simulink model "quadcopter_ex04_wind_test"  (R2025b)
settings: Solver=ode23t  StartTime=0.0  StopTime=timespot_spl(end)+2  FixedStep=0.01  MaxStep=1e-2  RelTol=1e-3  AbsTol=1e-3
PreLoadFcn:
  | [waypoints, timespot_spl, spline_data, spline_yaw, wayp_path_vis] = quadcopter_package_select_trajectory(2,true);
  | disp('Loaded path 2, round trip');
model workspace (MATLAB code in the model file):
  | load('xy_data_membrane.mat');
values from neighbouring files (symbols this model uses):
  wind_speed = 12    [quadcopter_ex04_wind_test_code.m]
undefined symbols (not defined in the file or in its folder): air_rho, battery_capacity, drone_leg, filtD_altitude, filtD_attitude, filtD_motor, filtD_position, filtD_yaw, filtM_altitude, filtM_attitude, filtM_position, filtM_yaw, filtSpd_motor, kd_altitude, kd_attitude, kd_motor, kd_position, kd_yaw, ki_altitude, ki_attitude, ki_motor, ki_position, ki_yaw, kp_altitude, kp_attitude, kp_motor, kp_position, kp_yaw, limit_altitude, limit_attitude, limit_motor, limit_yaw, pkgDensity, pkgSize, planedepth, pos2attitude, propeller, qc_motor, qd_area, qd_drag, spline_data, spline_yaw, timespot_spl, waypoints, X, Y, Z
libraries: sm_lib x77, nesl_utility x30, fl_lib x13, slpidlib x9, quadcopter_library x6, ee_lib x4, simulink x2, batteryecm_lib x1
(part 2 of 4)

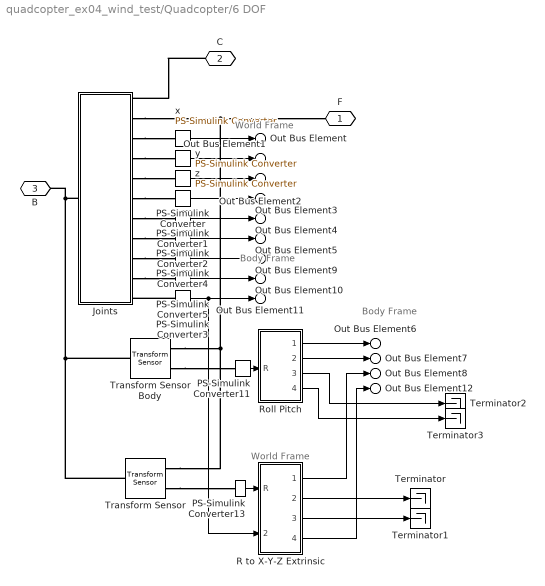
== system quadcopter_ex04_wind_test/Quadcopter/6 DOF ==
  note: Body Frame
  note: World Frame
  note: World Frame
  note: Body Frame
  Joints : Subsystem
  PS-Simulink Converter{,1..2,4..5} (5 alike) : nesl_utility/PS-Simulink Converter  PhysicalDomain=network_engine_domain  SubClassName=ps_output  LeftPortType=input  RightPortType=output  PseudoPeriodic=off  Frequencies=[]  VectorFormat=1-D array  Unit=inherit  AffineConversion=off
  PS-Simulink Converter11 : nesl_utility/PS-Simulink Converter  PhysicalDomain=network_engine_domain  SubClassName=ps_output  LeftPortType=input  RightPortType=output  PseudoPeriodic=off  Frequencies=[]  VectorFormat=1-D array  Unit=1  AffineConversion=off
  PS-Simulink Converter13 : nesl_utility/PS-Simulink Converter  PhysicalDomain=network_engine_domain  SubClassName=ps_output  LeftPortType=input  RightPortType=output  PseudoPeriodic=off  Frequencies=[]  VectorFormat=1-D array  Unit=1  AffineConversion=off
  PS-Simulink Converter3 : nesl_utility/PS-Simulink Converter  PhysicalDomain=network_engine_domain  SubClassName=ps_output  LeftPortType=input  RightPortType=output  PseudoPeriodic=off  Frequencies=[]  VectorFormat=1-D array  Unit=1  AffineConversion=off
  R to X-Y-Z Extrinsic : Subsystem  mask(Rotation Matrix to X-Y-Z Extrinsic){}
      mask help: Computes roll / pitch / yaw values assuming they correspond to X, Y, and Z rotations, applied in that order and using extrinsic rotations (rotations applied about the fixed axes of the base frame). Does not handle case where Y (pitch) rotation is +/-90 degrees.
  Roll Pitch : Subsystem
  Terminator{,1..3} (4 alike) : Terminator
  Transform Sensor : sm_lib/Frames and Transforms/Transform Sensor  MeasurementFrame=World  RotationSequence=XYX  SenseAngle=off  SenseAxis=off  SenseQ=off  SenseR=on  SenseRotationSequence=off  SenseOmegaX=off  SenseOmegaY=off  SenseOmegaZ=off  SenseOmega=off  SenseQDot=off  SenseRDot=off  SenseRotationSequenceDot=off  SenseAlphaX=off  SenseAlphaY=off  SenseAlphaZ=off  SenseAlpha=off  SenseQDDot=off  SenseRDDot=off  SenseX=off  SenseY=off  SenseZ=off  SenseXYZ=off  SenseRad=off  SenseAzim=off  SenseDist=off  SenseInc=off  SenseXDot=off  SenseYDot=off  SenseZDot=off  SenseXYZDot=off  SenseRadDot=off  SenseAzimDot=off  SenseDistDot=off  SenseIncDot=off  SenseXDDot=off  SenseYDDot=off  SenseZDDot=off  SenseXYZDDot=off  SenseRadDDot=off  SenseAzimDDot=off  SenseDistDDot=off  SenseIncDDot=off
  Transform Sensor Body : sm_lib/Frames and Transforms/Transform Sensor  MeasurementFrame=NonRotatingFollower  RotationSequence=XYX  SenseAngle=off  SenseAxis=off  SenseQ=off  SenseR=on  SenseRotationSequence=off  SenseOmegaX=off  SenseOmegaY=off  SenseOmegaZ=off  SenseOmega=off  SenseQDot=off  SenseRDot=off  SenseRotationSequenceDot=off  SenseAlphaX=off  SenseAlphaY=off  SenseAlphaZ=off  SenseAlpha=off  SenseQDDot=off  SenseRDDot=off  SenseX=off  SenseY=off  SenseZ=off  SenseXYZ=off  SenseRad=off  SenseAzim=off  SenseDist=off  SenseInc=off  SenseXDot=off  SenseYDot=off  SenseZDot=off  SenseXYZDot=off  SenseRadDot=off  SenseAzimDot=off  SenseDistDot=off  SenseIncDot=off  SenseXDDot=off  SenseYDDot=off  SenseZDDot=off  SenseXYZDDot=off  SenseRadDDot=off  SenseAzimDDot=off  SenseDistDDot=off  SenseIncDDot=off
  x : nesl_utility/PS-Simulink Converter  PhysicalDomain=network_engine_domain  SubClassName=ps_output  LeftPortType=input  RightPortType=output  PseudoPeriodic=off  Frequencies=[]  VectorFormat=1-D array  Unit=1  AffineConversion=off
  y : nesl_utility/PS-Simulink Converter  PhysicalDomain=network_engine_domain  SubClassName=ps_output  LeftPortType=input  RightPortType=output  PseudoPeriodic=off  Frequencies=[]  VectorFormat=1-D array  Unit=1  AffineConversion=off
  z : nesl_utility/PS-Simulink Converter  PhysicalDomain=network_engine_domain  SubClassName=ps_output  LeftPortType=input  RightPortType=output  PseudoPeriodic=off  Frequencies=[]  VectorFormat=1-D array  Unit=1  AffineConversion=off
  F : PMIOPort  Side=Left
  C : PMIOPort  Port=2  Side=Left
  B : PMIOPort  Port=3  Side=Left
  Out Bus Element : Outport  PortName=m  Element=px
  Out Bus Element1 : Outport  PortName=m  Element=vx
  Out Bus Element2 : Outport  PortName=m  Element=py
  Out Bus Element3 : Outport  PortName=m  Element=vy
  Out Bus Element4 : Outport  PortName=m  Element=pz
  Out Bus Element5 : Outport  PortName=m  Element=vz
  Out Bus Element6 : Outport  PortName=m  Element=roll
  Out Bus Element7 : Outport  PortName=m  Element=pitch
  Out Bus Element8 : Outport  PortName=m  Element=yaw
  Out Bus Element9 : Outport  PortName=m  Element=nRoll
  Out Bus Element10 : Outport  PortName=m  Element=nPitch
  Out Bus Element11 : Outport  PortName=m  Element=nYaw
  Out Bus Element12 : Outport  PortName=m  Element=yawWr
  wires:
  x/1 -> Out Bus Element/1
  y/1 -> Out Bus Element1/1
  R to X-Y-Z Extrinsic/1(yaw) -> Out Bus Element8/1
  PS-Simulink Converter1/1 -> Out Bus Element4/1
  PS-Simulink Converter2/1 -> Out Bus Element5/1
  z/1 -> Out Bus Element2/1
  PS-Simulink Converter/1 -> Out Bus Element3/1
  PS-Simulink Converter11/1 -> Roll Pitch/1(R)
  Roll Pitch/1(aRoll) -> Out Bus Element6/1
  Roll Pitch/2(aPitch) -> Out Bus Element7/1
  R to X-Y-Z Extrinsic/3(roll) -> Terminator1/1
  R to X-Y-Z Extrinsic/2(pitch) -> Terminator/1
  PS-Simulink Converter13/1 -> R to X-Y-Z Extrinsic/1(R)
  Roll Pitch/3(nRoll) -> Terminator2/1
  Roll Pitch/4(nPitch) -> Terminator3/1
  PS-Simulink Converter3/1 -> R to X-Y-Z Extrinsic/2(nYaw), Out Bus Element11/1
  PS-Simulink Converter4/1 -> Out Bus Element9/1
  PS-Simulink Converter5/1 -> Out Bus Element10/1
  R to X-Y-Z Extrinsic/4(yawWr) -> Out Bus Element12/1
  connections:
  Joints/RConn2 -- Transform Sensor/RConn1 -- Transform Sensor Body/RConn1 -- F/RConn1
  Joints/RConn3 -- x/LConn1
  Joints/RConn4 -- y/LConn1
  Transform Sensor Body/LConn1 -- Transform Sensor/LConn1 -- B/RConn1 -- Joints/LConn1
  Joints/RConn5 -- z/LConn1
  Joints/RConn6 -- PS-Simulink Converter/LConn1
  Joints/RConn7 -- PS-Simulink Converter1/LConn1
  Joints/RConn8 -- PS-Simulink Converter2/LConn1
  C/RConn1 -- Joints/RConn1
  Transform Sensor Body/RConn2 -- PS-Simulink Converter11/LConn1
  Transform Sensor/RConn2 -- PS-Simulink Converter13/LConn1
  PS-Simulink Converter3/LConn1 -- Joints/RConn11
  Joints/RConn9 -- PS-Simulink Converter4/LConn1
  Joints/RConn10 -- PS-Simulink Converter5/LConn1

== system quadcopter_ex04_wind_test/Quadcopter/Body ==
  " Arm2" : sm_lib/Body Elements/File Solid  ExtGeomFileName=quadcopter_drone_arm.stp  UnitType=FromFile  ExtGeomFileUnits=m  StepReaderType=HEX  ExportConvexHullGeometry=off  InertiaType=Custom  BasedOnType=Density  Density=1  DensityUnits=g/cm^3  Mass=0.0589152  MassUnits=kg  CenterOfMass=[-4.85019e-05, -0.00435236, -0.00536926]  CenterOfMassUnits=m  MomentsOfInertia=[0.000263222, 0.000260855, 1.23093e-05]  MomentsOfInertiaUnits=kg*m^2  ProductsOfInertia=[1.89459e-06, 5.49897e-08, 2.10429e-08]  ProductsOfInertiaUnits=kg*m^2  GraphicType=FromGeometry  MarkerShape=Sphere  MarkerSize=10  GraphicVisPropType=SimpleVisualProperties  GraphicDiffuseColor=[1.0 0.0 0.2]  GraphicOpacity=1.0  GraphicSpecularColor=[0.5 0.5 0.5 1.0]  GraphicAmbientColor=[0.15 0.15 0.15 1.0]  GraphicEmissiveColor=[0.0 0.0 0.0 1.0]  GraphicShininess=75  DoExposeReferenceFrame=off  SerializedFrames=<Frames><Frame><Id>Frame1</Id><Value><Name>port</Name><Origin><Source>GeometricFeature</Source><FeatureName>planar surface 13</FeatureName></Origin><PrimaryAxis><DefinedDirection>-Z</DefinedDirection><Source>ReferenceFrame</Source><SourceDirection>+Z</SourceDirection><FeatureName></FeatureName></PrimaryAxis><SecondaryAxis><DefinedDirection>-X</DefinedDirection><Source>ReferenceFrame</Source><SourceDirection>+X</SourceDirection><FeatureName></FeatureName></SecondaryAxis></Value></Frame><Frame><Id>Frame2</Id><Value><Name>F2</Name><Origin><Source>GeometricFeature</Source><FeatureName>planar surface 4</FeatureName></Origin><PrimaryAxis><DefinedDirection>+Z</DefinedDirection><Source>ReferenceFrame</Source><SourceDirection>+Z</SourceDirection><FeatureName></FeatureName></PrimaryAxis><SecondaryAxis><DefinedDirection>+X</DefinedDirection><Source>ReferenceFrame</Source><SourceDirection>+X</SourceDirection><FeatureName></FeatureName></SecondaryAxis></Value></Frame><Frame><Id>Frame4</Id><Value><Name>Foot</Name><Origin><Source>GeometricFeature</Source><FeatureName>planar surface 62</FeatureName></Origin><PrimaryAxis><DefinedDirection>+Z</DefinedDirection><Source>ReferenceFrame</Source><SourceDirection>+Z</SourceDirection><FeatureName></FeatureName></PrimaryAxis><SecondaryAxis><DefinedDirection>+X</DefinedDirection><Source>ReferenceFrame</Source><SourceDirection>+X</SourceDirection><FeatureName></FeatureName></SecondaryAxis></Value></Frame></Frames>
  " Arm4" : sm_lib/Body Elements/File Solid  ExtGeomFileName=quadcopter_drone_arm.stp  UnitType=FromFile  ExtGeomFileUnits=m  StepReaderType=HEX  ExportConvexHullGeometry=off  InertiaType=Custom  BasedOnType=Density  Density=1  DensityUnits=g/cm^3  Mass=0.0589152  MassUnits=kg  CenterOfMass=[-4.85019e-05, -0.00435236, -0.00536926]  CenterOfMassUnits=m  MomentsOfInertia=[0.000263222, 0.000260855, 1.23093e-05]  MomentsOfInertiaUnits=kg*m^2  ProductsOfInertia=[1.89459e-06, 5.49897e-08, 2.10429e-08]  ProductsOfInertiaUnits=kg*m^2  GraphicType=FromGeometry  MarkerShape=Sphere  MarkerSize=10  GraphicVisPropType=SimpleVisualProperties  GraphicDiffuseColor=[1.0 0.0 0.2]  GraphicOpacity=1.0  GraphicSpecularColor=[0.5 0.5 0.5 1.0]  GraphicAmbientColor=[0.15 0.15 0.15 1.0]  GraphicEmissiveColor=[0.0 0.0 0.0 1.0]  GraphicShininess=75  DoExposeReferenceFrame=off  SerializedFrames=<Frames><Frame><Id>Frame1</Id><Value><Name>port</Name><Origin><Source>GeometricFeature</Source><FeatureName>planar surface 13</FeatureName></Origin><PrimaryAxis><DefinedDirection>-Z</DefinedDirection><Source>ReferenceFrame</Source><SourceDirection>+Z</SourceDirection><FeatureName></FeatureName></PrimaryAxis><SecondaryAxis><DefinedDirection>-X</DefinedDirection><Source>ReferenceFrame</Source><SourceDirection>+X</SourceDirection><FeatureName></FeatureName></SecondaryAxis></Value></Frame><Frame><Id>Frame2</Id><Value><Name>F2</Name><Origin><Source>GeometricFeature</Source><FeatureName>planar surface 4</FeatureName></Origin><PrimaryAxis><DefinedDirection>+Z</DefinedDirection><Source>ReferenceFrame</Source><SourceDirection>+Z</SourceDirection><FeatureName></FeatureName></PrimaryAxis><SecondaryAxis><DefinedDirection>+X</DefinedDirection><Source>ReferenceFrame</Source><SourceDirection>+X</SourceDirection><FeatureName></FeatureName></SecondaryAxis></Value></Frame><Frame><Id>Frame3</Id><Value><Name>Foot</Name><Origin><Source>GeometricFeature</Source><FeatureName>planar surface 62</FeatureName></Origin><PrimaryAxis><DefinedDirection>+Z</DefinedDirection><Source>ReferenceFrame</Source><SourceDirection>+Z</SourceDirection><FeatureName></FeatureName></PrimaryAxis><SecondaryAxis><DefinedDirection>+X</DefinedDirection><Source>ReferenceFrame</Source><SourceDirection>+X</SourceDirection><FeatureName></FeatureName></SecondaryAxis></Value></Frame></Frames>
  Arm1 : sm_lib/Body Elements/File Solid  ExtGeomFileName=quadcopter_drone_arm.stp  UnitType=FromFile  ExtGeomFileUnits=m  StepReaderType=HEX  ExportConvexHullGeometry=off  InertiaType=Custom  BasedOnType=Density  Density=1  DensityUnits=g/cm^3  Mass=0.0589152  MassUnits=kg  CenterOfMass=[-4.85019e-05, -0.00435236, -0.00536926]  CenterOfMassUnits=m  MomentsOfInertia=[0.000263222, 0.000260855, 1.23093e-05]  MomentsOfInertiaUnits=kg*m^2  ProductsOfInertia=[1.89459e-06, 5.49897e-08, 2.10429e-08]  ProductsOfInertiaUnits=kg*m^2  GraphicType=FromGeometry  MarkerShape=Sphere  MarkerSize=10  GraphicVisPropType=SimpleVisualProperties  GraphicDiffuseColor=[1.0 1.0 1.0]  GraphicOpacity=1.0  GraphicSpecularColor=[0.5 0.5 0.5 1.0]  GraphicAmbientColor=[0.15 0.15 0.15 1.0]  GraphicEmissiveColor=[0.0 0.0 0.0 1.0]  GraphicShininess=75  DoExposeReferenceFrame=off  SerializedFrames=<Frames><Frame><Id>Frame1</Id><Value><Name>port</Name><Origin><Source>GeometricFeature</Source><FeatureName>planar surface 13</FeatureName></Origin><PrimaryAxis><DefinedDirection>-Z</DefinedDirection><Source>ReferenceFrame</Source><SourceDirection>+Z</SourceDirection><FeatureName></FeatureName></PrimaryAxis><SecondaryAxis><DefinedDirection>-X</DefinedDirection><Source>ReferenceFrame</Source><SourceDirection>+X</SourceDirection><FeatureName></FeatureName></SecondaryAxis></Value></Frame><Frame><Id>Frame2</Id><Value><Name>F2</Name><Origin><Source>GeometricFeature</Source><FeatureName>planar surface 4</FeatureName></Origin><PrimaryAxis><DefinedDirection>+Z</DefinedDirection><Source>ReferenceFrame</Source><SourceDirection>+Z</SourceDirection><FeatureName></FeatureName></PrimaryAxis><SecondaryAxis><DefinedDirection>+X</DefinedDirection><Source>ReferenceFrame</Source><SourceDirection>+X</SourceDirection><FeatureName></FeatureName></SecondaryAxis></Value></Frame><Frame><Id>Frame3</Id><Value><Name>Foot</Name><Origin><Source>GeometricFeature</Source><FeatureName>planar surface 62</FeatureName></Origin><PrimaryAxis><DefinedDirection>+Z</DefinedDirection><Source>ReferenceFrame</Source><SourceDirection>+Z</SourceDirection><FeatureName></FeatureName></PrimaryAxis><SecondaryAxis><DefinedDirection>+X</DefinedDirection><Source>ReferenceFrame</Source><SourceDirection>+X</SourceDirection><FeatureName></FeatureName></SecondaryAxis></Value></Frame></Frames>
  Arm3 : sm_lib/Body Elements/File Solid  ExtGeomFileName=quadcopter_drone_arm.stp  UnitType=FromFile  ExtGeomFileUnits=m  StepReaderType=HEX  ExportConvexHullGeometry=off  InertiaType=Custom  BasedOnType=Density  Density=1  DensityUnits=g/cm^3  Mass=0.0589152  MassUnits=kg  CenterOfMass=[-4.85019e-05, -0.00435236, -0.00536926]  CenterOfMassUnits=m  MomentsOfInertia=[0.000263222, 0.000260855, 1.23093e-05]  MomentsOfInertiaUnits=kg*m^2  ProductsOfInertia=[1.89459e-06, 5.49897e-08, 2.10429e-08]  ProductsOfInertiaUnits=kg*m^2  GraphicType=FromGeometry  MarkerShape=Sphere  MarkerSize=10  GraphicVisPropType=SimpleVisualProperties  GraphicDiffuseColor=[1.0 1.0 1.0]  GraphicOpacity=1.0  GraphicSpecularColor=[0.5 0.5 0.5 1.0]  GraphicAmbientColor=[0.15 0.15 0.15 1.0]  GraphicEmissiveColor=[0.0 0.0 0.0 1.0]  GraphicShininess=75  DoExposeReferenceFrame=off  SerializedFrames=<Frames><Frame><Id>Frame1</Id><Value><Name>port</Name><Origin><Source>GeometricFeature</Source><FeatureName>planar surface 13</FeatureName></Origin><PrimaryAxis><DefinedDirection>-Z</DefinedDirection><Source>ReferenceFrame</Source><SourceDirection>+Z</SourceDirection><FeatureName></FeatureName></PrimaryAxis><SecondaryAxis><DefinedDirection>-X</DefinedDirection><Source>ReferenceFrame</Source><SourceDirection>+X</SourceDirection><FeatureName></FeatureName></SecondaryAxis></Value></Frame><Frame><Id>Frame2</Id><Value><Name>F2</Name><Origin><Source>GeometricFeature</Source><FeatureName>planar surface 4</FeatureName></Origin><PrimaryAxis><DefinedDirection>+Z</DefinedDirection><Source>ReferenceFrame</Source><SourceDirection>+Z</SourceDirection><FeatureName></FeatureName></PrimaryAxis><SecondaryAxis><DefinedDirection>+X</DefinedDirection><Source>ReferenceFrame</Source><SourceDirection>+X</SourceDirection><FeatureName></FeatureName></SecondaryAxis></Value></Frame><Frame><Id>Frame3</Id><Value><Name>Foot</Name><Origin><Source>GeometricFeature</Source><FeatureName>planar surface 62</FeatureName></Origin><PrimaryAxis><DefinedDirection>+Z</DefinedDirection><Source>ReferenceFrame</Source><SourceDirection>+Z</SourceDirection><FeatureName></FeatureName></PrimaryAxis><SecondaryAxis><DefinedDirection>+X</DefinedDirection><Source>ReferenceFrame</Source><SourceDirection>+X</SourceDirection><FeatureName></FeatureName></SecondaryAxis></Value></Frame></Frames>
  Body : Subsystem
  Legs : Subsystem
  Transform Arm Ref : sm_lib/Frames and Transforms/Rigid Transform  RotationMethod=StandardAxis  FollAlignAxisA=+X  BaseAlignAxisA=+Y  FollAlignAxisB=+Y  BaseAlignAxisB=+Z  RotationStandardAxis=+Z  RotationAngle=45  RotationAngleUnits=deg  RotationArbitraryAxis=[0 0 1]  RotationSequenceAxes=FollowerAxes  RotationSequence=XYX  RotationSequenceAngles=[0 0 0]  RotationSequenceAnglesUnits=deg  RotationMatrix=[1 0 0; 0 1 0; 0 0 1]  Quaternion=[1 0 0 0]  TranslationMethod=Cartesian  TranslationCartesianOffset=[0 0 -26]  TranslationCartesianOffsetUnits=mm  TranslationStandardAxis=+Z  TranslationStandardOffset=0  TranslationStandardOffsetUnits=mm  TranslationROffset=0  TranslationROffsetUnits=m  TranslationThetaOffset=0  TranslationThetaOffsetUnits=deg  TranslationZOffset=0  TranslationZOffsetUnits=m
  Transform Arm1 : sm_lib/Frames and Transforms/Rigid Transform  RotationMethod=RotationSequence  FollAlignAxisA=+X  BaseAlignAxisA=+Y  FollAlignAxisB=+Y  BaseAlignAxisB=+Z  RotationStandardAxis=+Z  RotationAngle=0  RotationAngleUnits=deg  RotationArbitraryAxis=[0 0 1]  RotationSequenceAxes=FollowerAxes  RotationSequence=ZXZ  RotationSequenceAngles=[0 90 0]  RotationSequenceAnglesUnits=deg  RotationMatrix=[1 0 0; 0 1 0; 0 0 1]  Quaternion=[1 0 0 0]  TranslationMethod=Cartesian  TranslationCartesianOffset=[12 58 -38]  TranslationCartesianOffsetUnits=mm  TranslationStandardAxis=+Z  TranslationStandardOffset=0  TranslationStandardOffsetUnits=mm  TranslationROffset=0  TranslationROffsetUnits=m  TranslationThetaOffset=0  TranslationThetaOffsetUnits=deg  TranslationZOffset=0  TranslationZOffsetUnits=m
  Transform Arm2 : sm_lib/Frames and Transforms/Rigid Transform  RotationMethod=RotationSequence  FollAlignAxisA=+X  BaseAlignAxisA=+Y  FollAlignAxisB=+Y  BaseAlignAxisB=+Z  RotationStandardAxis=+Z  RotationAngle=-90  RotationAngleUnits=deg  RotationArbitraryAxis=[0 0 1]  RotationSequenceAxes=FollowerAxes  RotationSequence=ZXZ  RotationSequenceAngles=[-90 90 0]  RotationSequenceAnglesUnits=deg  RotationMatrix=[1 0 0; 0 1 0; 0 0 1]  Quaternion=[1 0 0 0]  TranslationMethod=Cartesian  TranslationCartesianOffset=[58 -12 -38]  TranslationCartesianOffsetUnits=mm  TranslationStandardAxis=+Z  TranslationStandardOffset=0  TranslationStandardOffsetUnits=mm  TranslationROffset=0  TranslationROffsetUnits=m  TranslationThetaOffset=0  TranslationThetaOffsetUnits=deg  TranslationZOffset=0  TranslationZOffsetUnits=m
  Transform Arm3 : sm_lib/Frames and Transforms/Rigid Transform  RotationMethod=RotationSequence  FollAlignAxisA=+X  BaseAlignAxisA=+Y  FollAlignAxisB=+Y  BaseAlignAxisB=+Z  RotationStandardAxis=+Z  RotationAngle=90  RotationAngleUnits=deg  RotationArbitraryAxis=[0 0 1]  RotationSequenceAxes=FollowerAxes  RotationSequence=ZXZ  RotationSequenceAngles=[90 90 0]  RotationSequenceAnglesUnits=deg  RotationMatrix=[1 0 0; 0 1 0; 0 0 1]  Quaternion=[1 0 0 0]  TranslationMethod=Cartesian  TranslationCartesianOffset=[-58 12 -38]  TranslationCartesianOffsetUnits=mm  TranslationStandardAxis=+Z  TranslationStandardOffset=0  TranslationStandardOffsetUnits=mm  TranslationROffset=0  TranslationROffsetUnits=m  TranslationThetaOffset=0  TranslationThetaOffsetUnits=deg  TranslationZOffset=0  TranslationZOffsetUnits=m
  Transform Arm4 : sm_lib/Frames and Transforms/Rigid Transform  RotationMethod=RotationSequence  FollAlignAxisA=+X  BaseAlignAxisA=+Y  FollAlignAxisB=+Y  BaseAlignAxisB=+Z  RotationStandardAxis=+Z  RotationAngle=180  RotationAngleUnits=deg  RotationArbitraryAxis=[0 0 1]  RotationSequenceAxes=FollowerAxes  RotationSequence=ZXZ  RotationSequenceAngles=[180 90 0]  RotationSequenceAnglesUnits=deg  RotationMatrix=[1 0 0; 0 1 0; 0 0 1]  Quaternion=[1 0 0 0]  TranslationMethod=Cartesian  TranslationCartesianOffset=[-12 -58 -38]  TranslationCartesianOffsetUnits=mm  TranslationStandardAxis=+Z  TranslationStandardOffset=0  TranslationStandardOffsetUnits=mm  TranslationROffset=0  TranslationROffsetUnits=m  TranslationThetaOffset=0  TranslationThetaOffsetUnits=deg  TranslationZOffset=0  TranslationZOffsetUnits=m
  P2 : PMIOPort  Side=Right
  "P1 " : PMIOPort  Port=2  Side=Left
  P3 : PMIOPort  Port=3  Side=Left
  P4 : PMIOPort  Port=4  Side=Right
  Ref : PMIOPort  Port=5  Side=Left
  G : PMIOPort  Port=6  Side=Right
  connections:
  Transform Arm4/LConn1 -- Transform Arm1/LConn1 -- Transform Arm3/LConn1 -- Transform Arm Ref/LConn1 -- Transform Arm2/LConn1
  Transform Arm4/RConn1 -- " Arm4"/LConn1
  " Arm2"/RConn1 -- P2/RConn1
  " Arm4"/RConn1 -- P4/RConn1
  Arm3/RConn1 -- P3/RConn1
  " Arm2"/LConn1 -- Transform Arm2/RConn1
  Transform Arm1/RConn1 -- Arm1/LConn1
  Arm1/RConn1 -- "P1 "/RConn1
  Arm3/LConn1 -- Transform Arm3/RConn1
  Legs/RConn1 -- G/RConn1
  Body/RConn1 -- Transform Arm Ref/RConn1
  Ref/RConn1 -- Legs/LConn1 -- Body/LConn1

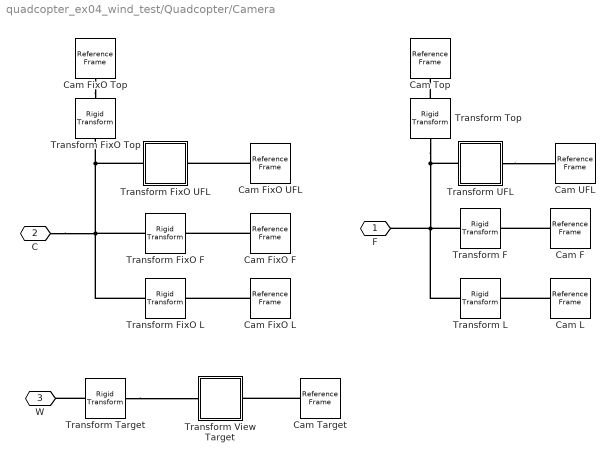
== system quadcopter_ex04_wind_test/Quadcopter/Camera ==
  Cam F : sm_lib/Frames and Transforms/Reference Frame
  Cam FixO F : sm_lib/Frames and Transforms/Reference Frame
  Cam FixO L : sm_lib/Frames and Transforms/Reference Frame
  Cam FixO Top : sm_lib/Frames and Transforms/Reference Frame
  Cam FixO UFL : sm_lib/Frames and Transforms/Reference Frame
  Cam L : sm_lib/Frames and Transforms/Reference Frame
  Cam Target : sm_lib/Frames and Transforms/Reference Frame
  Cam Top : sm_lib/Frames and Transforms/Reference Frame
  Cam UFL : sm_lib/Frames and Transforms/Reference Frame
  Transform Top : sm_lib/Frames and Transforms/Rigid Transform  RotationMethod=RotationSequence  FollAlignAxisA=+X  BaseAlignAxisA=+Y  FollAlignAxisB=+Y  BaseAlignAxisB=+Z  RotationStandardAxis=+Z  RotationAngle=0.0  RotationAngleUnits=deg  RotationArbitraryAxis=[0 0 1]  RotationSequenceAxes=FollowerAxes  RotationSequence=ZYX  RotationSequenceAngles=[0 90 0]  RotationSequenceAnglesUnits=deg  RotationMatrix=[1 0 0; 0 1 0; 0 0 1]  Quaternion=[1 0 0 0]  TranslationMethod=Cartesian  TranslationCartesianOffset=[0 0 1]  TranslationCartesianOffsetUnits=m  TranslationStandardAxis=+Z  TranslationStandardOffset=0  TranslationStandardOffsetUnits=m  TranslationROffset=0  TranslationROffsetUnits=m  TranslationThetaOffset=0  TranslationThetaOffsetUnits=deg  TranslationZOffset=0  TranslationZOffsetUnits=m
  Transform FixO Top : sm_lib/Frames and Transforms/Rigid Transform  RotationMethod=RotationSequence  FollAlignAxisA=+X  BaseAlignAxisA=+Y  FollAlignAxisB=+Y  BaseAlignAxisB=+Z  RotationStandardAxis=+Z  RotationAngle=0.0  RotationAngleUnits=deg  RotationArbitraryAxis=[0 0 1]  RotationSequenceAxes=FollowerAxes  RotationSequence=ZYX  RotationSequenceAngles=[0 90 0]  RotationSequenceAnglesUnits=deg  RotationMatrix=[1 0 0; 0 1 0; 0 0 1]  Quaternion=[1 0 0 0]  TranslationMethod=Cartesian  TranslationCartesianOffset=[0 0 1]  TranslationCartesianOffsetUnits=m  TranslationStandardAxis=+Z  TranslationStandardOffset=0  TranslationStandardOffsetUnits=m  TranslationROffset=0  TranslationROffsetUnits=m  TranslationThetaOffset=0  TranslationThetaOffsetUnits=deg  TranslationZOffset=0  TranslationZOffsetUnits=m
  Transform F : sm_lib/Frames and Transforms/Rigid Transform  RotationMethod=RotationSequence  FollAlignAxisA=+X  BaseAlignAxisA=+Y  FollAlignAxisB=+Y  BaseAlignAxisB=+Z  RotationStandardAxis=+Z  RotationAngle=0.0  RotationAngleUnits=deg  RotationArbitraryAxis=[0 0 1]  RotationSequenceAxes=FollowerAxes  RotationSequence=ZYX  RotationSequenceAngles=[180 0 0]  RotationSequenceAnglesUnits=deg  RotationMatrix=[1 0 0; 0 1 0; 0 0 1]  Quaternion=[1 0 0 0]  TranslationMethod=Cartesian  TranslationCartesianOffset=[1 0 0]  TranslationCartesianOffsetUnits=m  TranslationStandardAxis=+Z  TranslationStandardOffset=0  TranslationStandardOffsetUnits=m  TranslationROffset=0  TranslationROffsetUnits=m  TranslationThetaOffset=0  TranslationThetaOffsetUnits=deg  TranslationZOffset=0  TranslationZOffsetUnits=m
  Transform FixO F : sm_lib/Frames and Transforms/Rigid Transform  RotationMethod=RotationSequence  FollAlignAxisA=+X  BaseAlignAxisA=+Y  FollAlignAxisB=+Y  BaseAlignAxisB=+Z  RotationStandardAxis=+Z  RotationAngle=0.0  RotationAngleUnits=deg  RotationArbitraryAxis=[0 0 1]  RotationSequenceAxes=FollowerAxes  RotationSequence=ZYX  RotationSequenceAngles=[180 0 0]  RotationSequenceAnglesUnits=deg  RotationMatrix=[1 0 0; 0 1 0; 0 0 1]  Quaternion=[1 0 0 0]  TranslationMethod=Cartesian  TranslationCartesianOffset=[1 0 0]  TranslationCartesianOffsetUnits=m  TranslationStandardAxis=+Z  TranslationStandardOffset=0  TranslationStandardOffsetUnits=m  TranslationROffset=0  TranslationROffsetUnits=m  TranslationThetaOffset=0  TranslationThetaOffsetUnits=deg  TranslationZOffset=0  TranslationZOffsetUnits=m
  Transform FixO L : sm_lib/Frames and Transforms/Rigid Transform  RotationMethod=RotationSequence  FollAlignAxisA=+X  BaseAlignAxisA=+Y  FollAlignAxisB=+Y  BaseAlignAxisB=+Z  RotationStandardAxis=+Z  RotationAngle=0.0  RotationAngleUnits=deg  RotationArbitraryAxis=[0 0 1]  RotationSequenceAxes=FollowerAxes  RotationSequence=ZYX  RotationSequenceAngles=[90 0 0]  RotationSequenceAnglesUnits=deg  RotationMatrix=[1 0 0; 0 1 0; 0 0 1]  Quaternion=[1 0 0 0]  TranslationMethod=Cartesian  TranslationCartesianOffset=[0 -1 0]  TranslationCartesianOffsetUnits=m  TranslationStandardAxis=+Z  TranslationStandardOffset=0  TranslationStandardOffsetUnits=m  TranslationROffset=0  TranslationROffsetUnits=m  TranslationThetaOffset=0  TranslationThetaOffsetUnits=deg  TranslationZOffset=0  TranslationZOffsetUnits=m
  Transform FixO UFL : Subsystem  mask{offset_xyz=[0.5 -1 1]}
      mask prompts: offset_xyz "Offset [x y z] (m)"
      mask init:
      | seq_zyx_follower = [atan2d(-offset_xyz(2),-offset_xyz(1)) atan2d(offset_xyz(3),sqrt(offset_xyz(1)^2+offset_xyz(2)^2)) 0];
  Transform L : sm_lib/Frames and Transforms/Rigid Transform  RotationMethod=RotationSequence  FollAlignAxisA=+X  BaseAlignAxisA=+Y  FollAlignAxisB=+Y  BaseAlignAxisB=+Z  RotationStandardAxis=+Z  RotationAngle=0.0  RotationAngleUnits=deg  RotationArbitraryAxis=[0 0 1]  RotationSequenceAxes=FollowerAxes  RotationSequence=ZYX  RotationSequenceAngles=[90 0 0]  RotationSequenceAnglesUnits=deg  RotationMatrix=[1 0 0; 0 1 0; 0 0 1]  Quaternion=[1 0 0 0]  TranslationMethod=Cartesian  TranslationCartesianOffset=[0 -1 0]  TranslationCartesianOffsetUnits=m  TranslationStandardAxis=+Z  TranslationStandardOffset=0  TranslationStandardOffsetUnits=m  TranslationROffset=0  TranslationROffsetUnits=m  TranslationThetaOffset=0  TranslationThetaOffsetUnits=deg  TranslationZOffset=0  TranslationZOffsetUnits=m
  Transform Target : sm_lib/Frames and Transforms/Rigid Transform  RotationMethod=None  FollAlignAxisA=+X  BaseAlignAxisA=+Y  FollAlignAxisB=+Y  BaseAlignAxisB=+Z  RotationStandardAxis=+Z  RotationAngle=0.0  RotationAngleUnits=deg  RotationArbitraryAxis=[0 0 1]  RotationSequenceAxes=FollowerAxes  RotationSequence=ZYX  RotationSequenceAngles=[90 0 0]  RotationSequenceAnglesUnits=deg  RotationMatrix=[1 0 0; 0 1 0; 0 0 1]  Quaternion=[1 0 0 0]  TranslationMethod=Cartesian  TranslationCartesianOffset=[waypoints(1:2,end)' 0 ]  TranslationCartesianOffsetUnits=m  TranslationStandardAxis=+Z  TranslationStandardOffset=0  TranslationStandardOffsetUnits=m  TranslationROffset=0  TranslationROffsetUnits=m  TranslationThetaOffset=0  TranslationThetaOffsetUnits=deg  TranslationZOffset=0  TranslationZOffsetUnits=m
  Transform UFL : Subsystem  mask{offset_xyz=[0.5 -1 1]}
      mask prompts: offset_xyz "Offset [x y z] (m)"
      mask init:
      | seq_zyx_follower = [atan2d(-offset_xyz(2),-offset_xyz(1)) atan2d(offset_xyz(3),sqrt(offset_xyz(1)^2+offset_xyz(2)^2)) 0];
  Transform View Target : Subsystem  mask{offset_xyz=[1.5 -1.5 1]}
      mask prompts: offset_xyz "Offset [x y z] (m)"
      mask init:
      | seq_zyx_follower = [atan2d(-offset_xyz(2),-offset_xyz(1)) atan2d(offset_xyz(3),sqrt(offset_xyz(1)^2+offset_xyz(2)^2)) 0];
  F : PMIOPort  Side=Right
  C : PMIOPort  Port=2  Side=Right
  W : PMIOPort  Port=3  Side=Right
  connections:
  Transform Top/LConn1 -- Transform UFL/LConn1 -- F/RConn1 -- Transform F/LConn1 -- Transform L/LConn1
  C/RConn1 -- Transform FixO L/LConn1 -- Transform FixO F/LConn1 -- Transform FixO UFL/LConn1 -- Transform FixO Top/LConn1
  Cam FixO Top/RConn1 -- Transform FixO Top/RConn1
  Transform Top/RConn1 -- Cam Top/RConn1
  Cam FixO L/RConn1 -- Transform FixO L/RConn1
  Cam L/RConn1 -- Transform L/RConn1
  Cam FixO F/RConn1 -- Transform FixO F/RConn1
  Cam F/RConn1 -- Transform F/RConn1
  Transform UFL/RConn1 -- Cam UFL/RConn1
  Cam FixO UFL/RConn1 -- Transform FixO UFL/RConn1
  Transform Target/LConn1 -- W/RConn1
  Transform Target/RConn1 -- Transform View Target/LConn1
  Cam Target/RConn1 -- Transform View Target/RConn1

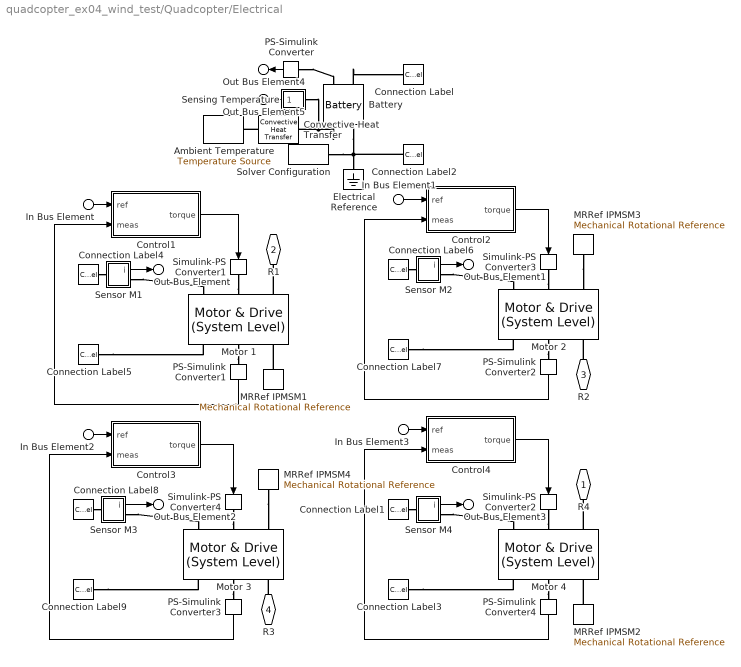
== system quadcopter_ex04_wind_test/Quadcopter/Electrical ==
  In Bus Element : Inport  PortName=cmd  Element=w1
  In Bus Element1 : Inport  PortName=cmd  Element=w2
  In Bus Element2 : Inport  PortName=cmd  Element=w3
  In Bus Element3 : Inport  PortName=cmd  Element=w4
  Ambient Temperature : fl_lib/Thermal/Thermal Sources/Temperature Source  temperature=air_temperature K
  Battery : batteryecm_lib/Battery  Vnom=14 V  prm_dir=1  R1_dis=2 Ohm  R1_ch=2 Ohm  R1=2e-2 Ohm  prm_AH=2  AH=battery_capacity A*hr  V1=11.5 V  AH1=battery_capacity/2 A*hr  prm_R2=1  R2=2000 Ohm  Tmeas=298.15 K  charge_measurement_port=simscape.enum.battery.enable.yes  prm_dyn=1  Rp1=0.005 Ohm  tau1=30 s  Rp2=0.005 Ohm  tau2=30 s  Rp3=0.005 Ohm  tau3=30 s  Rp4=0.005 Ohm  tau4=30 s  Rp5=0.005 Ohm  tau5=30 s  prm_fade=1  N_fade=100  AH_fade=45 A*hr  R1_fade=2.02 Ohm  R1_ch_fade=2.02 Ohm  V1_fade=10.35 V  prm_age=1  prm_age_OCV=1  OCV_age=0.9  SOC_age=60  Tmeas_age=298.15 K  delta_time_age_vec=[0] d  temperature_age_vec=[273] K  OCV_scaling_age=2.2134e6  OCV_offset_age=1.632e6  temp_exp_age=0.515833569 V  t_exp_age=0.75  Vnom_T2=12 V  R1_T2=2e-2 Ohm  R1_T2_dis=2.2 Ohm  R1_T2_ch=2.2 Ohm  V1_T2=11.4 V  R2_T2=2200 Ohm  Rp1_T2=0.005 Ohm  tau1_T2=30 s  Rp2_T2=0.005 Ohm  tau2_T2=30 s  Rp3_T2=0.005 Ohm  tau3_T2=30 s  Rp4_T2=0.005 Ohm  tau4_T2=30 s  Rp5_T2=0.005 Ohm  tau5_T2=30 s  Tmeas2=273.15 K  thermal_port=simscape.enum.thermaleffects.model  thermal_mass=30000 J/K  i_specify=off  i_priority=None  i=0 A  i_nominal_specify=off  i_nominal_value=1  i_nominal_unit=A  v_specify=off  v_priority=None  v=0 V  v_nominal_specify=off  v_nominal_value=1  v_nominal_unit=V  charge_specify=on  charge_priority=High  charge=battery_capacity A*hr  charge_nominal_specify=off  charge_nominal_value=1  charge_nominal_unit=A*hr  num_cycles_specify=off  num_cycles_priority=High  num_cycles=0  num_cycles_nominal_specify=off  num_cycles_nominal_value=1  num_cycles_nominal_unit=1  temperature_specify=on  temperature_priority=High  temperature=air_temperature K  temperature_nominal_specify=off  temperature_nominal_value=1  temperature_nominal_unit=K
      settings: InternalSimscapePortConfiguration="{\"Bottom\":[],\"Left\":[{\"id\":\"p\",\"label\":\"+\",\"type\":\"foundation.electrical.electrical\"},{\"id\":\"q\",\"label\":\"q\",\"type\":\"output\"}],\"Right\":[{\"id\":\"n\",\"label\":\"-\",\"type\":\"foundation.electrical.electrical\"},{\"id\":\"H\",\"label\":\"H\",\"type\":\"foundation.thermal.thermal\"}],\"Top\":[]}"
  Connection Label{,1,4,6,8} (5 alike) : ConnectionLabel  Label=p
  Connection Label{2..3,5,7,9} (5 alike) : ConnectionLabel  Label=n
  Control1 : Subsystem
  Control2 : Subsystem
  Control3 : Subsystem
  Control4 : Subsystem
  Convective Heat Transfer : fl_lib/Thermal/Thermal Elements/Convective Heat Transfer  thermal_type=foundation.enum.constant_variable.constant  area=3e-3 m^2  heat_tr_coeff=20 W/(m^2*K)  min_heat_tr_coeff=1e-3 W/(K*m^2)  T_specify=off  T_priority=None  T=0 K  T_nominal_specify=off  T_nominal_value=1  T_nominal_unit=K  Q_specify=off  Q_priority=None  Q=0 W  Q_nominal_specify=off  Q_nominal_value=1  Q_nominal_unit=W
  Electrical Reference : fl_lib/Electrical/Electrical Elements/Electrical Reference
  MRRef IPMSM{1..4} (4 alike) : fl_lib/Mechanical/Rotational Elements/Mechanical Rotational Reference
  Motor {1..4} (4 alike) : ee_lib/Electromechanical/Motor & Drive (System Level)  torque_speed_param=ee.enum.electromech.envelope.torque_power  overtorque_param=ee.enum.electromech.overtorque.no  T_t=[.09, .08, .07, 0] N*m  T_t_intermittent=[.36, .32, .28, 0] N*m  T_t_2D=[.09, .09, .09; .08, .08, .08; .07, .07, .07; 0, 0, 0] N*m  T_t_intermittent_2D=[.36, .36, .36; .32, .32, .32; .28, .28, .28; 0, 0, 0] N*m  w_t=[0, 3750, 7500, 8000] rpm  vdc_t=[6, 12, 24] V  torque_max=trq_max N*m  power_max=power_max W  torque_max_intermittent=0.4 N*m  power_max_intermittent=120 W  time_overtorque=30 s  time_recover=60 s  Tc=trq_tc s  EnableSwitch=simscape.enum.onoff.off  losses_param=1  eff=eff_overall  w_eff=eff_spd rpm  T_eff=eff_trq N*m  Piron=0 % not important in first iteration W  Pbase=0 % not important in first iteration W  w_eff_vec=[-8000, -4000, 0, 4000, 8000] rpm  T_eff_vec=[0, .03, .06, .09] N*m  v_eff_vec=[100, 250, 400] V  losses_mat=[1.49, 1.67, 2.21, 3.1; .42, .69, 1.14, 2.03; .06, .24, .78, 1.68; .42, .69, 1.14, 2.03; 1.49, 1.67, 2.21, 3.1] W  efficiency_mat=[95, 95, 95, 95; 95, 95, 95, 95; 95, 95, 95, 95; 95, 95, 95, 95; 95, 95, 95, 95]  losses_mat_3D=ones(5, 4, 3) W  efficiency_mat_3D=95 * ones(5, 4, 3)  Res=0 % not important in first iteration Ohm  J=0 kg*m^2  lam=rotor_d N*m/(rad/s)  speed0=0 rpm  faulted_specify=off  faulted_priority=None  faulted=0  faulted_nominal_specify=off  faulted_nominal_value=1  faulted_nominal_unit=1  isSwitchedOff_specify=off  isSwitchedOff_priority=None  isSwitchedOff=0  isSwitchedOff_nominal_specify=off  isSwitchedOff_nominal_value=1  isSwitchedOff_nominal_unit=1  torqueLimitContinuous_specify=off  torqueLimitContinuous_priority=None  torqueLimitContinuous=0 N*m  torqueLimitContinuous_nominal_specify=off  torqueLimitContinuous_nominal_value=1  torqueLimitContinuous_nominal_unit=N*m  alpha=3.93e-3 1/K  Tmeas=25 degC  Tmeas2=125 degC  losses_mat_T2=[1.49, 1.74, 2.49, 3.74; .42, .67, 1.42, 2.67; .06, .31, 1.06, 2.31; .42, .67, 1.42, 2.67; 1.49, 1.74, 2.49, 3.74] W  efficiency_mat_T2=[95, 95, 95, 95; 95, 95, 95, 95; 95, 95, 95, 95; 95, 95, 95, 95; 95, 95, 95, 95]  losses_mat_3D_T2=ones(5, 4, 3) W  efficiency_mat_3D_T2=95 * ones(5, 4, 3)  thermal_mass=100 J/K  initial_temperature=25 degC
  PS-Simulink Converter : nesl_utility/PS-Simulink Converter  PhysicalDomain=network_engine_domain  SubClassName=ps_output  LeftPortType=input  RightPortType=output  PseudoPeriodic=off  Frequencies=[]  VectorFormat=1-D array  Unit=hr*A  AffineConversion=off
  PS-Simulink Converter{1..4} (4 alike) : nesl_utility/PS-Simulink Converter  PhysicalDomain=network_engine_domain  SubClassName=ps_output  LeftPortType=input  RightPortType=output  PseudoPeriodic=off  Frequencies=[]  VectorFormat=1-D array  Unit=rpm  AffineConversion=off
  Sensing Temperature : Subsystem
  Sensor M1 : Subsystem
      mask Display: disp('i');
  Sensor M2 : Subsystem
      mask Display: disp('i');
  Sensor M3 : Subsystem
      mask Display: disp('i');
  Sensor M4 : Subsystem
      mask Display: disp('i');
  Simulink-PS Converter{1..4} (4 alike) : nesl_utility/Simulink-PS Converter  PhysicalDomain=network_engine_domain  SubClassName=ps_input  LeftPortType=input  RightPortType=output  PseudoPeriodic=off  Frequencies=[]  NoiseDistribution=none  NoiseParameters=[]  Unit=N*m  AffineConversion=off  FilteringAndDerivatives=provide  SimscapeFilterOrder=1  InputFilterTimeConstant=0.001  UdotUserProvided=0
  Solver Configuration : nesl_utility/Solver Configuration  PhysicalDomain=network_engine_domain  SubClassName=solver  LeftPortType=input  RightPortType=generic  Tones=[]  Harmonics=[]  SimulateNoise=off  Profile=off  UseLocalSampling=off  EnableSwitchedLinearOptims=on  FrequencyDomain=off  UseCCode=off  RelTol=0.001  AbsTol=1e-06  MinStep=1e-09  ToWorkspace=off  RevertToSquareIcSolve=off  NumHomotopyIterations=100  PhasorMode=off  PhasorModeNumHarmonics=1  ConsistencySolver=NEWTON_FTOL  IndexReductionMethod=DerivativeReplacement  DoDC=off  ResidualTolerance=1e-9  ConsistencyTolSource=GLOBAL  ConsistencyAbsTol=0.001  ConsistencyRelTol=0.001  ConsistencyTolFactor=0.001  UseLocalSolver=off  LocalSolverChoice=NE_BACKWARD_EULER_ADVANCER  ResolveIndetEquations=on  FunctionEvalNumThread=1  LocalSolverSampleTime=0.01  DoFixedCost=off  MaxNonlinIter=2  MaxModeIter=2  ComputeImpulses=off  ImpulseIterations=2  LinearAlgebra=auto  LinearAlgebraNumThread=0  EquationFormulation=NE_TIME_EF  DelaysMemoryBudget=1024  AutomaticFiltering=on  FilteringTimeConstant=0.001  PartitionStorageMethod=AS_NEEDED  PartitionMemoryBudget=1024  PartitionMethod=FAST  MultibodyUseLocalSolver=off  MultibodyLocalSolverChoice=ODE1  MultibodyLocalSolverSampleTime=0.001
  R4 : PMIOPort  Side=Left
  R1 : PMIOPort  Port=2  Side=Right
  R2 : PMIOPort  Port=3  Side=Left
  R3 : PMIOPort  Port=4  Side=Right
  Out Bus Element : Outport  PortName=m  Element=Mot1.i
  Out Bus Element1 : Outport  PortName=m  Element=Mot2.i
  Out Bus Element2 : Outport  PortName=m  Element=Mot3.i
  Out Bus Element3 : Outport  PortName=m  Element=Mot4.i
  Out Bus Element5 : Outport  PortName=m  Element=Battery.degC
  Out Bus Element4 : Outport  PortName=m  Element=Battery.SOC
  wires:
  In Bus Element3/1 -> Control4/1(ref)
  Sensor M4/1(i) -> Out Bus Element3/1
  Sensor M1/1(i) -> Out Bus Element/1
  In Bus Element/1 -> Control1/1(ref)
  In Bus Element1/1 -> Control2/1(ref)
  Sensor M2/1(i) -> Out Bus Element1/1
  Sensor M3/1(i) -> Out Bus Element2/1
  In Bus Element2/1 -> Control3/1(ref)
  Control2/1(torque) -> Simulink-PS Converter3/1
  Control1/1(torque) -> Simulink-PS Converter1/1
  Control3/1(torque) -> Simulink-PS Converter4/1
  Control4/1(torque) -> Simulink-PS Converter2/1
  PS-Simulink Converter/1 -> Out Bus Element4/1
  Sensing Temperature/1(T) -> Out Bus Element5/1
  PS-Simulink Converter2/1 -> Control2/2(meas)
  PS-Simulink Converter1/1 -> Control1/2(meas)
  PS-Simulink Converter3/1 -> Control3/2(meas)
  PS-Simulink Converter4/1 -> Control4/2(meas)
  connections:
  Connection Label2/LConn1 -- Battery/RConn1 -- Solver Configuration/RConn1 -- Electrical Reference/LConn1
  Battery/LConn1 -- Connection Label/LConn1
  MRRef IPMSM2/LConn1 -- Motor 4/RConn3
  Simulink-PS Converter2/RConn1 -- Motor 4/LConn2
  Motor 4/RConn2 -- PS-Simulink Converter4/LConn1
  Motor 4/LConn3 -- R4/RConn1
  Connection Label3/LConn1 -- Motor 4/RConn1
  Connection Label1/LConn1 -- Sensor M4/LConn1
  Sensor M4/RConn1 -- Motor 4/LConn1
  Sensor M1/RConn1 -- Motor 1/LConn1
  Connection Label5/LConn1 -- Motor 1/RConn1
  Motor 1/LConn3 -- R1/RConn1
  Simulink-PS Converter1/RConn1 -- Motor 1/LConn2
  MRRef IPMSM1/LConn1 -- Motor 1/RConn3
  Motor 1/RConn2 -- PS-Simulink Converter1/LConn1
  Connection Label4/LConn1 -- Sensor M1/LConn1
  Connection Label6/LConn1 -- Sensor M2/LConn1
  Motor 2/RConn2 -- PS-Simulink Converter2/LConn1
  MRRef IPMSM3/LConn1 -- Motor 2/LConn3
  Simulink-PS Converter3/RConn1 -- Motor 2/LConn2
  Connection Label7/LConn1 -- Motor 2/RConn1
  R2/RConn1 -- Motor 2/RConn3
  Sensor M2/RConn1 -- Motor 2/LConn1
  Sensor M3/RConn1 -- Motor 3/LConn1
  R3/RConn1 -- Motor 3/RConn3
  Simulink-PS Converter4/RConn1 -- Motor 3/LConn2
  MRRef IPMSM4/LConn1 -- Motor 3/LConn3
  Motor 3/RConn2 -- PS-Simulink Converter3/LConn1
  Connection Label8/LConn1 -- Sensor M3/LConn1
  Connection Label9/LConn1 -- Motor 3/RConn1
  PS-Simulink Converter/LConn1 -- Battery/LConn2
  Battery/RConn2 -- Sensing Temperature/LConn1 -- Convective Heat Transfer/LConn1
  Convective Heat Transfer/RConn1 -- Ambient Temperature/LConn1

== system quadcopter_ex04_wind_test/Quadcopter/Ground ==
  Ground : Subsystem  mask{waypoints=waypoints}
      mask prompts: waypoints "Waypoints [xyz] (m)"
      mask init:
      | plane_x = max(waypoints(1,:))-min(waypoints(1,:))+6;
      | plane_y = max(waypoints(2,:))-min(waypoints(2,:))+6;
      | 
      | offset_x = plane_x/2+min(waypoints(1,:))-3;
      | offset_y = plane_y/2+min(waypoints(2,:))-3;
  Infinite Plane : sm_lib/Curves and Surfaces/Infinite Plane  GraphicType=None  GraphicPlaneWidth=1  GraphicPlaneWidthUnits=m  GraphicPlaneHeight=1  GraphicPlaneHeightUnits=m  GraphicVisPropType=SimpleVisualProperties  GraphicDiffuseColor=[0.5 0.5 0.5]  GraphicOpacity=0  GraphicSpecularColor=[0.5 0.5 0.5 1.0]  GraphicAmbientColor=[0.15 0.15 0.15 1.0]  GraphicEmissiveColor=[0.0 0.0 0.0 1.0]  GraphicShininess=75
  Launch Insignia : sm_lib/Body Elements/Extruded Solid  ExtrusionType=General  PolygonNumSides=3  PolygonOuterRadius=1  PolygonOuterRadiusUnits=m  ExportEntireGeometry=off  ExtrusionCrossSection=[0.15 0.15; -0.15 0.15; -0.15 0.75; -0.6 0.75; -0.6 -0.75; -0.15 -0.75; -0.15 -0.15; 0.15 -0.15; 0.15 -0.75; 0.6 -0.75; 0.6 0.75; 0.15 0.75]*0.5  ExtrusionCrossSectionUnits=m  ExportConvexHullGeometry=off  ExtrusionLength=0.002  ExtrusionLengthUnits=m  InertiaType=CalculateFromGeometry  BasedOnType=Density  Density=1  DensityUnits=kg/m^3  Mass=1  MassUnits=kg  CenterOfMass=[0 0 0]  CenterOfMassUnits=m  MomentsOfInertia=[1 1 1]  MomentsOfInertiaUnits=kg*m^2  ProductsOfInertia=[0 0 0]  ProductsOfInertiaUnits=kg*m^2  GraphicType=FromGeometry  MarkerShape=Sphere  MarkerSize=10  GraphicVisPropType=SimpleVisualProperties  GraphicDiffuseColor=[0.3 0.3 0.3]  GraphicOpacity=1.0  GraphicSpecularColor=[0.5 0.5 0.5 1.0]  GraphicAmbientColor=[0.15 0.15 0.15 1.0]  GraphicEmissiveColor=[0.0 0.0 0.0 1.0]  GraphicShininess=75  DoExposeReferenceFrame=on  SerializedFrames=<Frames/>
  Launch Ring : sm_lib/Body Elements/Revolved Solid  RevolutionCrossSection=[0.5 0.001; 0.5 -0.001; 0.75 -0.001; 0.75 0.001]  RevolutionCrossSectionUnits=m  RevolutionExtent=Full  RevolutionAngle=180  RevolutionAngleUnits=deg  ExportConvexHullGeometry=off  InertiaType=CalculateFromGeometry  BasedOnType=Density  Density=1000  DensityUnits=kg/m^3  Mass=1  MassUnits=kg  CenterOfMass=[0 0 0]  CenterOfMassUnits=m  MomentsOfInertia=[1 1 1]  MomentsOfInertiaUnits=kg*m^2  ProductsOfInertia=[0 0 0]  ProductsOfInertiaUnits=kg*m^2  GraphicType=FromGeometry  MarkerShape=Sphere  MarkerSize=10  GraphicVisPropType=SimpleVisualProperties  GraphicDiffuseColor=[0.3 0.3 0.3]  GraphicOpacity=1.0  GraphicSpecularColor=[0.5 0.5 0.5 1.0]  GraphicAmbientColor=[0.15 0.15 0.15 1.0]  GraphicEmissiveColor=[0.0 0.0 0.0 1.0]  GraphicShininess=75  DoExposeReferenceFrame=on  SerializedFrames=<Frames/>
  Target Inner Ring : sm_lib/Body Elements/Revolved Solid  RevolutionCrossSection=[0.5 0.001; 0.5 -0.001; 0.75 -0.001; 0.75 0.001]*0.25  RevolutionCrossSectionUnits=m  RevolutionExtent=Full  RevolutionAngle=180  RevolutionAngleUnits=deg  ExportConvexHullGeometry=off  InertiaType=CalculateFromGeometry  BasedOnType=Density  Density=1000  DensityUnits=kg/m^3  Mass=1  MassUnits=kg  CenterOfMass=[0 0 0]  CenterOfMassUnits=m  MomentsOfInertia=[1 1 1]  MomentsOfInertiaUnits=kg*m^2  ProductsOfInertia=[0 0 0]  ProductsOfInertiaUnits=kg*m^2  GraphicType=FromGeometry  MarkerShape=Sphere  MarkerSize=10  GraphicVisPropType=SimpleVisualProperties  GraphicDiffuseColor=[1.0 0.2 0.2]  GraphicOpacity=1.0  GraphicSpecularColor=[0.5 0.5 0.5 1.0]  GraphicAmbientColor=[0.15 0.15 0.15 1.0]  GraphicEmissiveColor=[0.0 0.0 0.0 1.0]  GraphicShininess=75  DoExposeReferenceFrame=on  SerializedFrames=<Frames/>
  Target Middle Ring : sm_lib/Body Elements/Revolved Solid  RevolutionCrossSection=[0.5 0.001; 0.5 -0.001; 0.75 -0.001; 0.75 0.001]*0.5  RevolutionCrossSectionUnits=m  RevolutionExtent=Full  RevolutionAngle=180  RevolutionAngleUnits=deg  ExportConvexHullGeometry=off  InertiaType=CalculateFromGeometry  BasedOnType=Density  Density=1000  DensityUnits=kg/m^3  Mass=1  MassUnits=kg  CenterOfMass=[0 0 0]  CenterOfMassUnits=m  MomentsOfInertia=[1 1 1]  MomentsOfInertiaUnits=kg*m^2  ProductsOfInertia=[0 0 0]  ProductsOfInertiaUnits=kg*m^2  GraphicType=FromGeometry  MarkerShape=Sphere  MarkerSize=10  GraphicVisPropType=SimpleVisualProperties  GraphicDiffuseColor=[1.0 0.8 0.2]  GraphicOpacity=1.0  GraphicSpecularColor=[0.5 0.5 0.5 1.0]  GraphicAmbientColor=[0.15 0.15 0.15 1.0]  GraphicEmissiveColor=[0.0 0.0 0.0 1.0]  GraphicShininess=75  DoExposeReferenceFrame=on  SerializedFrames=<Frames/>
  Target Outer Ring : sm_lib/Body Elements/Revolved Solid  RevolutionCrossSection=[0.5 0.001; 0.5 -0.001; 0.75 -0.001; 0.75 0.001]  RevolutionCrossSectionUnits=m  RevolutionExtent=Full  RevolutionAngle=180  RevolutionAngleUnits=deg  ExportConvexHullGeometry=off  InertiaType=CalculateFromGeometry  BasedOnType=Density  Density=1000  DensityUnits=kg/m^3  Mass=1  MassUnits=kg  CenterOfMass=[0 0 0]  CenterOfMassUnits=m  MomentsOfInertia=[1 1 1]  MomentsOfInertiaUnits=kg*m^2  ProductsOfInertia=[0 0 0]  ProductsOfInertiaUnits=kg*m^2  GraphicType=FromGeometry  MarkerShape=Sphere  MarkerSize=10  GraphicVisPropType=SimpleVisualProperties  GraphicDiffuseColor=[0.2 0.4 1.0]  GraphicOpacity=1.0  GraphicSpecularColor=[0.5 0.5 0.5 1.0]  GraphicAmbientColor=[0.15 0.15 0.15 1.0]  GraphicEmissiveColor=[0.0 0.0 0.0 1.0]  GraphicShininess=75  DoExposeReferenceFrame=on  SerializedFrames=<Frames/>
  Trajectory : Subsystem
  Transform Launch : sm_lib/Frames and Transforms/Rigid Transform  RotationMethod=None  FollAlignAxisA=+X  BaseAlignAxisA=+Y  FollAlignAxisB=+Y  BaseAlignAxisB=+Z  RotationStandardAxis=+Z  RotationAngle=0.0  RotationAngleUnits=deg  RotationArbitraryAxis=[0 0 1]  RotationSequenceAxes=FollowerAxes  RotationSequence=XYX  RotationSequenceAngles=[0 0 0]  RotationSequenceAnglesUnits=deg  RotationMatrix=[1 0 0; 0 1 0; 0 0 1]  Quaternion=[1 0 0 0]  TranslationMethod=Cartesian  TranslationCartesianOffset=[waypoints(1:2,1)' 0 ]  TranslationCartesianOffsetUnits=m  TranslationStandardAxis=+Z  TranslationStandardOffset=0  TranslationStandardOffsetUnits=m  TranslationROffset=0  TranslationROffsetUnits=m  TranslationThetaOffset=0  TranslationThetaOffsetUnits=deg  TranslationZOffset=0  TranslationZOffsetUnits=m
  Transform Target : sm_lib/Frames and Transforms/Rigid Transform  RotationMethod=None  FollAlignAxisA=+X  BaseAlignAxisA=+Y  FollAlignAxisB=+Y  BaseAlignAxisB=+Z  RotationStandardAxis=+Z  RotationAngle=0.0  RotationAngleUnits=deg  RotationArbitraryAxis=[0 0 1]  RotationSequenceAxes=FollowerAxes  RotationSequence=XYX  RotationSequenceAngles=[0 0 0]  RotationSequenceAnglesUnits=deg  RotationMatrix=[1 0 0; 0 1 0; 0 0 1]  Quaternion=[1 0 0 0]  TranslationMethod=Cartesian  TranslationCartesianOffset=[waypoints(1:2,end)' 0 ]  TranslationCartesianOffsetUnits=m  TranslationStandardAxis=+Z  TranslationStandardOffset=0  TranslationStandardOffsetUnits=m  TranslationROffset=0  TranslationROffsetUnits=m  TranslationThetaOffset=0  TranslationThetaOffsetUnits=deg  TranslationZOffset=0  TranslationZOffsetUnits=m
  W : PMIOPort  Side=Right
  G : PMIOPort  Port=2  Side=Left
  connections:
  Launch Insignia/RConn1 -- Launch Ring/RConn1 -- Transform Launch/RConn1
  W/RConn1 -- Ground/LConn1 -- Transform Launch/LConn1 -- Transform Target/LConn1 -- Trajectory/RConn1
  Target Middle Ring/RConn1 -- Target Inner Ring/RConn1 -- Transform Target/RConn1 -- Target Outer Ring/RConn1
  Infinite Plane/LConn1 -- Ground/RConn1
  Infinite Plane/RConn1 -- G/RConn1
